simulink model "mod_08"  (R2025a)
settings: Solver=ode45  StartTime=0.0  StopTime=20  MaxStep=1e-2  RelTol=1e-3
values from neighbouring files (symbols this model uses):
  o = z*w    (= -6)    [res_transitoria.m]
  w = 3    [res_transitoria.m]
settings Model: Creator=fabri  LastModifiedBy=fabri

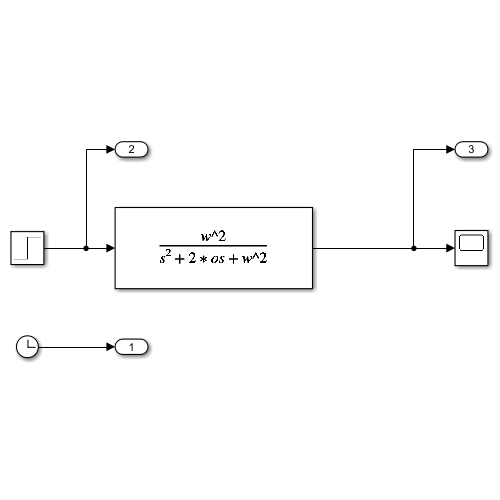
[thumbnail: Simulink's stored preview of the top-level diagram]
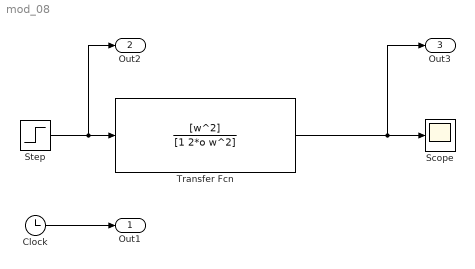
== system mod_08 ==
  Clock : Clock
  Scope : Scope
      settings: ActiveDisplayYMinimum=-3.3274442522775  ActiveDisplayYMaximum=8.7743430671098182
  Step : Step  Time=0  SampleTime=0
  Transfer Fcn : TransferFcn  Numerator=[w^2]  Denominator=[1 2*o w^2]
  Out1 : Outport
  Out2 : Outport  Port=2
  Out3 : Outport  Port=3
  wires:
  Step/1 -> Out2/1, Transfer Fcn/1
  Transfer Fcn/1 -> Out3/1, Scope/1
  Clock/1 -> Out1/1
